simulink model "pm"  (R2023b)
settings: Solver=VariableStepAuto  StartTime=0.0  StopTime=0.1  MaxStep=1e-8  RelTol=1e-3
settings Model: Creator=user  LastModifiedBy=user

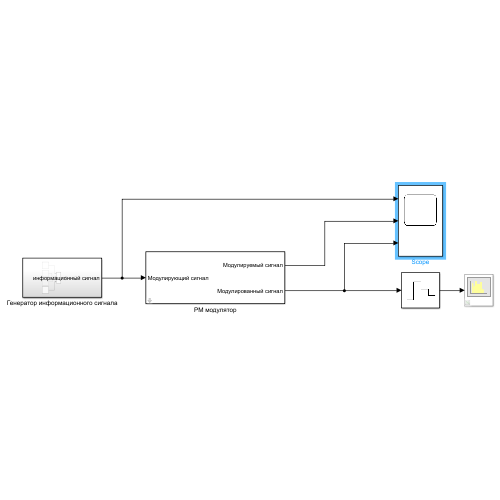
[thumbnail: Simulink's stored preview of the top-level diagram]
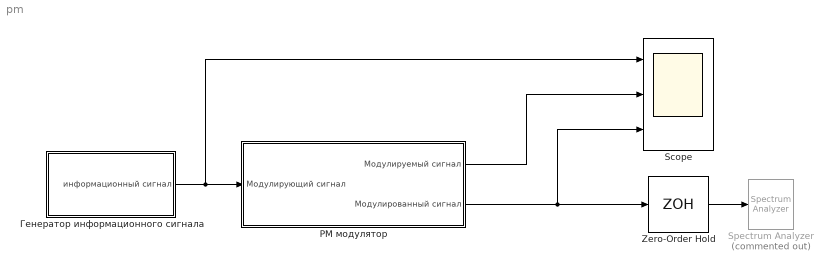
== system pm ==
  PM модулятор : Subsystem  mask{freq=1000, m=2*pi}
      mask prompts: freq "Частота несущей"; m "Девиция фазы"
  Scope : Scope  NumInputPorts=3
  Spectrum Analyzer : SpectrumAnalyzer  Commented=on  WindowPosition=[439.000000,257.000000,800.000000,500.000000,]  ScopeFrameLocation=window  SampleRateSource=Property  SampleRate=1000  PlotAsTwoSidedSpectrum=off  StartFrequency=20  StopFrequency=20e3  YLimits=[-179.88994486,-8.65773485]  SelectedToolstripTab=spectrumAnalyzerToolstrip.estimationTab
  Zero-Order Hold : ZeroOrderHold  SampleTime=1e-3
  Генератор информационного сигнала : Subsystem
  wires:
  Генератор информационного сигнала/1(информационный сигнал) -> Scope/1, PM модулятор/1(Модулирующий сигнал)
  Zero-Order Hold/1 -> Spectrum Analyzer/1
  PM модулятор/2(Модулированный сигнал) -> Scope/3, Zero-Order Hold/1
  PM модулятор/1(Модулируемый сигнал) -> Scope/2

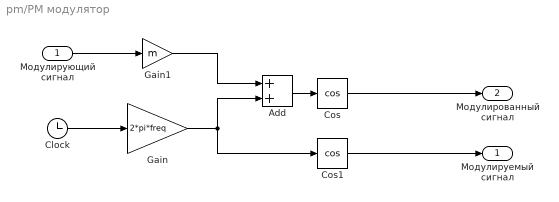
== system pm/PM модулятор ==
  Модулирующий сигнал : Inport
  Add : Sum
  Clock : Clock
  Cos : Trigonometry  Operator=cos
  Cos1 : Trigonometry  Operator=cos
  Gain : Gain  Gain=2*pi*freq
  Gain1 : Gain  Gain=m
  Модулируемый сигнал : Outport
  Модулированный сигнал : Outport  Port=2
  wires:
  Clock/1 -> Gain/1
  Модулирующий сигнал/1 -> Gain1/1
  Add/1 -> Cos/1
  Gain/1 -> Cos1/1, Add/2
  Gain1/1 -> Add/1
  Cos/1 -> Модулированный сигнал/1
  Cos1/1 -> Модулируемый сигнал/1

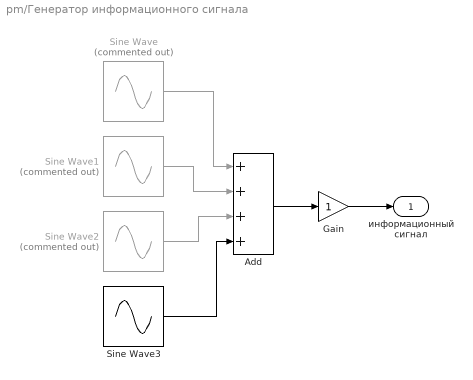
== system pm/Генератор информационного сигнала ==
  Add : Sum  Inputs=++++
  Gain : Gain
  Sine Wave : Sin  Commented=on  Frequency=40*2*pi  SampleTime=0
  Sine Wave1 : Sin  Commented=on  Frequency=60*2*pi  SampleTime=0
  Sine Wave2 : Sin  Commented=on  Frequency=80*2*pi  SampleTime=0
  Sine Wave3 : Sin  Frequency=100*2*pi  SampleTime=0
  информационный сигнал : Outport
  wires:
  Sine Wave1/1 -> Add/2
  Sine Wave2/1 -> Add/3
  Sine Wave3/1 -> Add/4
  Sine Wave/1 -> Add/1
  Add/1 -> Gain/1
  Gain/1 -> информационный сигнал/1
